simulink model "ClarkeParkTest"  (R2026a)
settings: Solver=FixedStepDiscrete  StopTime=ctCfg.Duration  FixedStep=ctCfg.Ts
PostLoadFcn:
  | addpath(fullfile(fileparts(get_param('ClarkeParkTest','FileName')),'..','build_process')); initialize_clarke_park_test('ClarkeParkTest');
model workspace (MAT data in the model file):
  ctCfg.Ts = 0.0001
  ctCfg.Duration = 0.1
  ctCfg.Amplitude = 5
  ctCfg.FrequencyHz = 50
  ctCfg.InitialAngleRad = 0.3
  ctCfg.AngleOffsetRad = 0
  ctCfg.UseIndependentInverse = 0
  ctCfg.ZeroSequenceGain = 1
  ctCfg.RandomSeed = 2026
  ctStim.time = []
  ctStim.signals.values = [4.77668244563 4.72791287112 4.67447741741 4.61642881885 4.5538243624 4.48672583108 4.41519944307 4.33931578625 4.25914974865 4.17478044445 4.08629113599 3.99376915152 ... (7007 elements, 1001x7)]
  ctStim.signals.dimensions = 7
libraries: ClarkePark x4
settings Model: Creator=24322  LastModifiedBy=24322

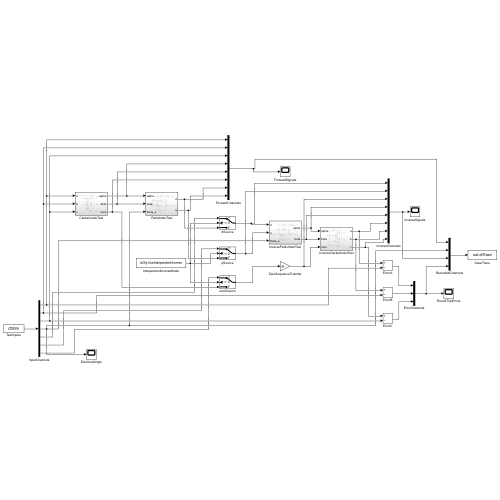
[thumbnail: Simulink's stored preview of the top-level diagram]
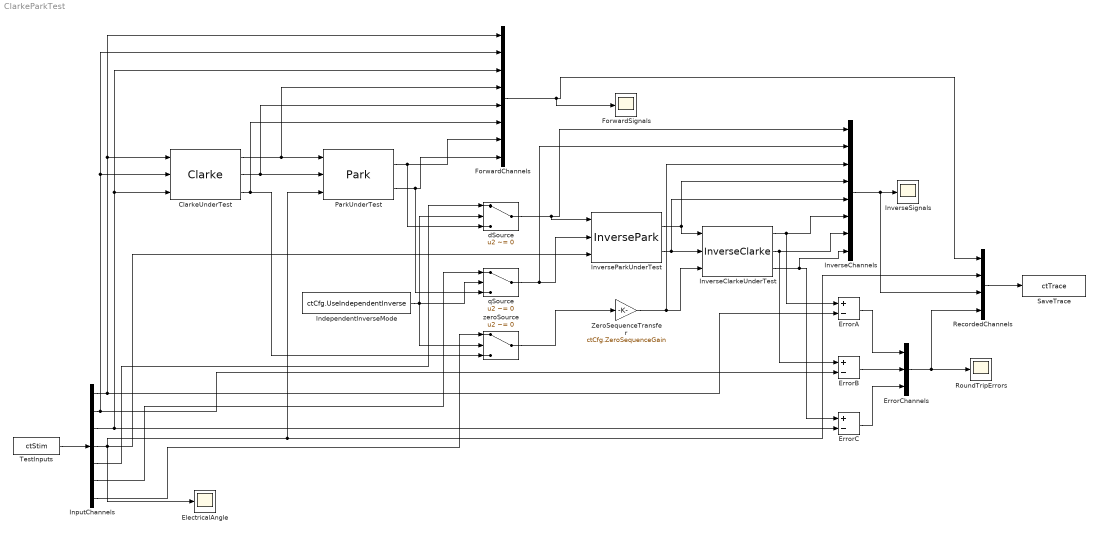
== system ClarkeParkTest ==
  ClarkeUnderTest : ClarkePark/Clarke  SystemSampleTime=-1  VariantActivationTime=update diagram  EmptyChoice=off  PassThrough=off  PassThroughVariantControl=(default)  EmptyChoiceVariantControl=(default)  AllowFlexibleInterface=on  Latency=0  AutoFrameSizeCalculation=off
  ElectricalAngle : Scope
      settings: Title=Electrical angle  YLabel=rad
  ErrorA : Sum  Inputs=+-
  ErrorB : Sum  Inputs=+-
  ErrorC : Sum  Inputs=+-
  ErrorChannels : Mux  Inputs=3
  ForwardChannels : Mux  Inputs=8
  ForwardSignals : Scope
      settings: Title=Forward: abc / alpha-beta-zero / dq  ActiveDisplayYMinimum=-6.2499617609940312  ActiveDisplayYMaximum=6.2499957512215651  YLabel=A
  IndependentInverseMode : Constant  Value=ctCfg.UseIndependentInverse
  InputChannels : Demux  Outputs=7
  InverseChannels : Mux  Inputs=8
  InverseClarkeUnderTest : ClarkePark/InverseClarke  SystemSampleTime=-1  VariantActivationTime=update diagram  EmptyChoice=off  PassThrough=off  PassThroughVariantControl=(default)  EmptyChoiceVariantControl=(default)  AllowFlexibleInterface=on  Latency=0  AutoFrameSizeCalculation=off
  InverseParkUnderTest : ClarkePark/InversePark  SystemSampleTime=-1  VariantActivationTime=update diagram  EmptyChoice=off  PassThrough=off  PassThroughVariantControl=(default)  EmptyChoiceVariantControl=(default)  AllowFlexibleInterface=on  Latency=0  AutoFrameSizeCalculation=off
  InverseSignals : Scope
      settings: Title=Inverse: selected dq0 / alpha-beta / abc  YLabel=A
  ParkUnderTest : ClarkePark/Park  SystemSampleTime=-1  VariantActivationTime=update diagram  EmptyChoice=off  PassThrough=off  PassThroughVariantControl=(default)  EmptyChoiceVariantControl=(default)  AllowFlexibleInterface=on  Latency=0  AutoFrameSizeCalculation=off
  RecordedChannels : Mux
  RoundTripErrors : Scope
      settings: Title=Reconstructed minus original (round-trip mode)  YLabel=A
  SaveTrace : ToWorkspace  VariableName=ctTrace  SaveFormat=Structure With Time  SampleTime=-1
  TestInputs : FromWorkspace  VariableName=ctStim  SampleTime=ctCfg.Ts  Interpolate=off  OutputAfterFinalValue=Holding final value
  ZeroSequenceTransfer : Gain  Gain=ctCfg.ZeroSequenceGain
  dSource : Switch  Criteria=u2 ~= 0  SaturateOnIntegerOverflow=off  InputSameDT=off
  qSource : Switch  Criteria=u2 ~= 0  SaturateOnIntegerOverflow=off  InputSameDT=off
  zeroSource : Switch  Criteria=u2 ~= 0  SaturateOnIntegerOverflow=off  InputSameDT=off
  wires:
  RecordedChannels/1 -> SaveTrace/1
  ErrorChannels/1 -> RecordedChannels/4, RoundTripErrors/1
  InverseChannels/1 -> RecordedChannels/3, InverseSignals/1
  ForwardChannels/1 -> RecordedChannels/1, ForwardSignals/1
  ErrorC/1 -> ErrorChannels/3
  ErrorB/1 -> ErrorChannels/2
  ErrorA/1 -> ErrorChannels/1
  InverseClarkeUnderTest/3 -> InverseChannels/8, ErrorC/1
  InverseClarkeUnderTest/2 -> InverseChannels/7, ErrorB/1
  InverseClarkeUnderTest/1 -> InverseChannels/6, ErrorA/1
  ZeroSequenceTransfer/1 -> InverseClarkeUnderTest/3, InverseChannels/3
  InverseParkUnderTest/2 -> InverseClarkeUnderTest/2, InverseChannels/5
  InverseParkUnderTest/1 -> InverseClarkeUnderTest/1, InverseChannels/4
  zeroSource/1 -> ZeroSequenceTransfer/1
  qSource/1 -> InverseParkUnderTest/2, InverseChannels/2
  dSource/1 -> InverseParkUnderTest/1, InverseChannels/1
  ClarkeUnderTest/3 -> ForwardChannels/6, zeroSource/3
  InputChannels/7 -> zeroSource/1
  ParkUnderTest/2 -> qSource/3, ForwardChannels/8
  InputChannels/6 -> qSource/1
  ParkUnderTest/1 -> dSource/3, ForwardChannels/7
  IndependentInverseMode/1 -> dSource/2, qSource/2, zeroSource/2
  InputChannels/5 -> dSource/1
  InputChannels/4 -> ParkUnderTest/3, RecordedChannels/2, InverseParkUnderTest/3, ElectricalAngle/1
  ClarkeUnderTest/2 -> ForwardChannels/5, ParkUnderTest/2
  ClarkeUnderTest/1 -> ParkUnderTest/1, ForwardChannels/4
  InputChannels/3 -> ClarkeUnderTest/3, ForwardChannels/3, ErrorC/2
  InputChannels/2 -> ClarkeUnderTest/2, ForwardChannels/2, ErrorB/2
  InputChannels/1 -> ClarkeUnderTest/1, ForwardChannels/1, ErrorA/2
  TestInputs/1 -> InputChannels/1
